simulink model "bpsk_cdm_carrier_lpf_waveform"  (R2025b)
settings: Solver=FixedStepAuto  StartTime=0.0  StopTime=50/6.2e6  MaxStep=3.33e-9  RelTol=1e-3
undefined symbols (not defined in the file): K, wc
libraries: commseqgen3 x4, commfilt2 x3, dspstat3 x2, commchan3 x1, commdigbbndpm3 x1, commrandsrc3 x1
settings Model: Creator=trish  LastModifiedBy=axolotl

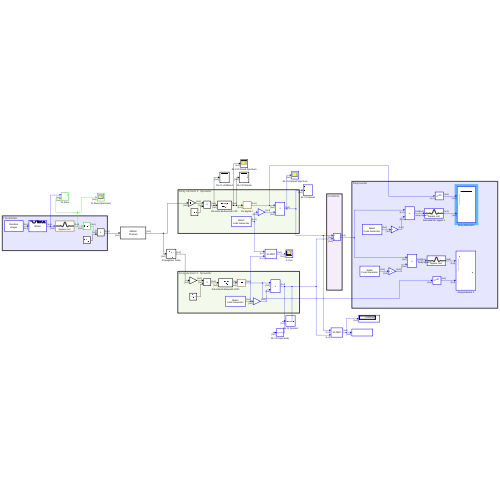
[thumbnail: Simulink's stored preview of the top-level diagram]
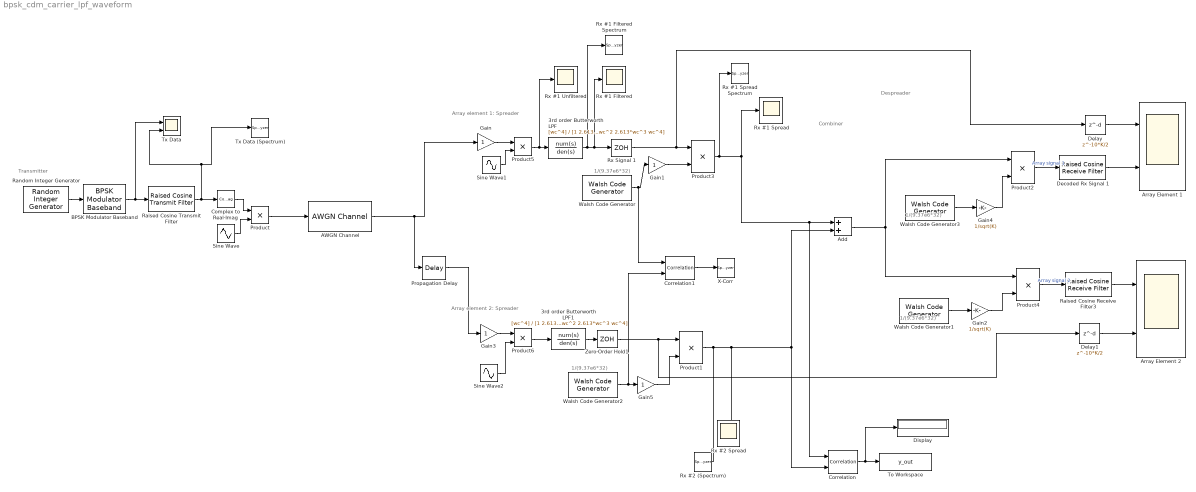
== system bpsk_cdm_carrier_lpf_waveform ==
  note: Despreader
  note: Combiner
  note: 1/(9.37e6*32)
  note: Array element 1: Spreader
  note: Transmitter
  note: 1/(9.37e6*32)
  note: 1/(9.37e6*32)
  note: Array element 2: Spreader
  note: 1/(9.37e6*32)
  3rd order Butterworth LPF : TransferFcn  Numerator=[wc^4]  Denominator=[1 2.613*wc 3.414*wc^2 2.613*wc^3 wc^4]
  3rd order Butterworth LPF1 : TransferFcn  Numerator=[wc^4]  Denominator=[1 2.613*wc 3.414*wc^2 2.613*wc^3 wc^4]
  AWGN Channel : commchan3/AWGN Channel  LegacyMode=off  NoiseMethod="Signal to noise ratio  (SNR)"  noiseMode="Signal to noise ratio  (SNR)"  EbNo=10  EsNo=10  SNR=10  BitsPerSymbol=1  SignalPower=1  SpecifySymbolPeriod=off  SamplesPerSymbol=1  SymbolPeriod=1  VarianceSource=Parameter  Variance=1  RandomStream=mt19937ar with seed  Seed=67  SimulateUsing=Code generation
  Add : Sum
  Array Element 1 : Scope  NumInputPorts=2
      settings: ActiveDisplayYMinimum=-0.22565656393453695  ActiveDisplayYMaximum=0.20472975996592438  DataLoggingVariableName=ScopeData7
  Array Element 2 : Scope  NumInputPorts=2
      settings: TimeUnits=Metric (based on Time Span)  ActiveDisplayYMinimum=-0.25790948055422058  ActiveDisplayYMaximum=0.25862522470755545  YLabel=Amplitude  DataLoggingVariableName=ScopeData2
  BPSK Modulator Baseband : commdigbbndpm3/BPSK Modulator Baseband  Ph=0  outDtype=double  outWordLen=16  outUDDataType=sfix(16)  outFracLenMode=Best precision  outFracLen=15  outDataTypeStr=double  outLastDataTypeStr=double
  Complex to Real-Imag : ComplexToRealImag  Output=Real
  Correlation : dspstat3/Correlation  domain=Time  roundingMode=Floor  overflowMode=off  outputDataTypeStr=Inherit: Same as accumulator  outputMin=[]  outputMax=[]  outputLastDataTypeStr=Inherit: Same as accumulator
  Correlation1 : dspstat3/Correlation  domain=Time  roundingMode=Floor  overflowMode=off  outputDataTypeStr=Inherit: Same as accumulator  outputMin=[]  outputMax=[]  outputLastDataTypeStr=Inherit: Same as accumulator
  Decoded Rx Signal 1 : commfilt2/Raised Cosine Receive Filter  filtType=Square root  R=0.5  filtSpan=10  N=K  downFactor=1  downOffset=0  filterGain=1  RateOptions=Allow multirate processing  framing=Mute  checkCoeff=off  variableName=rcRxFilt2  currentFiltSpan=10  D=5  inputOffset=0  sampMode=Mute  saveAsFlag=0  rateMode=Downsampling  checkGain=Normalized  launchFVT=on  roundingMode=Floor  overflowMode=off  coeffDataTypeStr=Inherit: Same word length as input  coeffMin=[]  coeffMax=[]  coeffLastDataTypeStr=Inherit: Same word length as input  accumDataTypeStr=Inherit: Same as product output  accumLastDataTypeStr=Inherit: Same as product output  outputDataTypeStr=Inherit: Same as accumulator  outputMin=[]  outputMax=[]  outputLastDataTypeStr=Inherit: Same as accumulator
  Delay : Delay  DelayLength=10*K/2
  Delay1 : Delay  DelayLength=10*K/2
  Display : Display
  Gain{,1,3,5} (4 alike) : Gain
  Gain2 : Gain  Gain=1/sqrt(K)
  Gain4 : Gain  Gain=1/sqrt(K)
  Product{,1..6} (7 alike) : Product
  Propagation Delay : TransportDelay  DelayTime=2e-9  TransDelayFeedthrough=on
  Raised Cosine Receive Filter3 : commfilt2/Raised Cosine Receive Filter  filtType=Square root  R=0.5  filtSpan=10  N=K  downFactor=1  downOffset=0  filterGain=1  RateOptions=Allow multirate processing  framing=Mute  checkCoeff=off  variableName=rcRxFilt3  currentFiltSpan=10  D=5  inputOffset=0  sampMode=Mute  saveAsFlag=0  rateMode=Downsampling  checkGain=Normalized  launchFVT=on  roundingMode=Floor  overflowMode=off  coeffDataTypeStr=Inherit: Same word length as input  coeffMin=[]  coeffMax=[]  coeffLastDataTypeStr=Inherit: Same word length as input  accumDataTypeStr=Inherit: Same as product output  accumLastDataTypeStr=Inherit: Same as product output  outputDataTypeStr=Inherit: Same as accumulator  outputMin=[]  outputMax=[]  outputLastDataTypeStr=Inherit: Same as accumulator
  Raised Cosine Transmit Filter : commfilt2/Raised Cosine Transmit Filter  filtType=Square root  R=0.5  filtSpan=10  N=K*5  filterGain=1  RateOptions=Allow multirate processing  framing=Mute  checkCoeff=off  variableName=rcTxFilt  checkGain=Normalized  sampMode=Mute  saveAsFlag=0  currentFiltSpan=10  D=5  launchFVT=on  roundingMode=Floor  overflowMode=off  coeffDataTypeStr=Inherit: Same word length as input  coeffMin=[]  coeffMax=[]  coeffLastDataTypeStr=Inherit: Same word length as input  outputDataTypeStr=Inherit: Same as accumulator  outputMin=[]  outputMax=[]  outputLastDataTypeStr=Inherit: Same as accumulator
      settings: LibrarySourceBlock=|
      | commhdlfilt/Raised Cosine
      | Transmit Filter
  Random Integer Generator : commrandsrc3/Random Integer Generator  SetSize=2  SeedSource=Parameter  Seed=32  SampleTime=1/(6.25e6)  SamplesPerFrame=1  OutputDataType=single  SimulateUsing=Interpreted execution
  Rx #1 Filtered : Scope
      settings: TimeUnits=Metric (based on Time Span)  ActiveDisplayYMinimum=-0.50683787517471779  ActiveDisplayYMaximum=0.55095946181705846  YLabel=Amplitude  DataLoggingVariableName=ScopeData4
  Rx #1 Filtered Spectrum : SpectrumAnalyzer  WindowPosition=[133.000000,75.000000,2748.000000,1782.000000,]  ScopeFrameLocation=window  SpectrumType=Power density  Method=Welch  WindowInvariantSamplesPerUpdate=on  Span=300e6  StartFrequency=-25000000  StopFrequency=25000000  SpectrumUnits=dBm/Hz  YLimits=[-331.5621 29.6853]  ExpandToolstrip=on  SelectedToolstripTab=spectrumAnalyzerToolstrip.estimationTab
      settings: OpenAtSimulationStart=off
  Rx #1 Spread : Scope
      settings: TimeUnits=Metric (based on Time Span)  ActiveDisplayYMinimum=-0.38058083882507643  ActiveDisplayYMaximum=0.3711759796363393  YLabel=Amplitude  DataLoggingVariableName=ScopeData3
  Rx #1 Spread Spectrum : SpectrumAnalyzer  WindowPosition=[89.000000,50.000000,1832.000000,1188.000000,]  ScopeFrameLocation=window  SpectrumType=Power density  Method=Welch  WindowInvariantSamplesPerUpdate=on  Span=300e6  StartFrequency=-25000000  StopFrequency=25000000  SpectrumUnits=dBm/Hz  YLimits=[-148.08026488239346 -43.11631661926841]  ExpandToolstrip=on  SelectedToolstripTab=spectrumAnalyzerToolstrip.estimationTab
      settings: OpenAtSimulationStart=off
  Rx #1 Unfiltered : Scope
      settings: TimeUnits=Metric (based on Time Span)  ActiveDisplayYMinimum=-4.3884399589650158  ActiveDisplayYMaximum=5.1372737935889194  YLabel=Amplitude  DataLoggingVariableName=ScopeData6
  Rx #2 (Spectrum) : SpectrumAnalyzer  WindowPosition=[149.000000,75.000000,2732.000000,1782.000000,]  ScopeFrameLocation=window  SpectrumType=Power density  Method=Welch  WindowInvariantSamplesPerUpdate=on  Span=300e6  StartFrequency=-25000000  StopFrequency=25000000  SpectrumUnits=dBm/Hz  YLimits=[-151.3459 -44.247]  ExpandToolstrip=on  SelectedToolstripTab=spectrumAnalyzerToolstrip.estimationTab
      settings: OpenAtSimulationStart=off
  Rx #2 Spread : Scope
      settings: TimeUnits=Metric (based on Time Span)  ActiveDisplayYMinimum=-0.38058083882507643  ActiveDisplayYMaximum=0.3711759796363393  YLabel=Amplitude
  Rx Signal 1 : ZeroOrderHold  SampleTime=1/(K*9.35e6)
  Sine Wave : Sin  Frequency=2*pi*500e6  Phase=pi/2  SampleTime=0
  Sine Wave1 : Sin  Frequency=2*pi*500e6  Phase=pi/2  SampleTime=0
  Sine Wave2 : Sin  Frequency=2*pi*500e6  Phase=pi/2  SampleTime=0
  To Workspace : ToWorkspace  VariableName=y_out  SampleTime=-1
      settings: Save2DSignal=2-D array (concatenate along first dimension)
  Tx Data : Scope  NumInputPorts=2
      settings: ActiveDisplayYMinimum=-1.25  ActiveDisplayYMaximum=1.25
  Tx Data (Spectrum) : SpectrumAnalyzer  WindowPosition=[4261.000000,672.000000,1832.000000,1188.000000,]  ScopeFrameLocation=window  SpectrumType=Power density  Method=Welch  WindowInvariantSamplesPerUpdate=on  Span=60e6  StartFrequency=-25000000  StopFrequency=25000000  SpectrumUnits=dBm/Hz  YLimits=[-129.66030778637997 -44.78293119034885]  ExpandToolstrip=on  SelectedToolstripTab=spectrumAnalyzerToolstrip.estimationTab
      settings: OpenAtSimulationStart=off
  Walsh Code Generator : commseqgen3/Walsh Code Generator  Length=K  Index=1  SampleTime=1/(K*9.35e6)  SamplesPerFrame=1  OutputDataType=int8  SimulateUsing=Code generation
  Walsh Code Generator1 : commseqgen3/Walsh Code Generator  Length=K  Index=2  SampleTime=1/(K*9.35e6)  SamplesPerFrame=1  OutputDataType=double  SimulateUsing=Code generation
  Walsh Code Generator2 : commseqgen3/Walsh Code Generator  Length=K  Index=2  SampleTime=1/(K*9.35e6)  SamplesPerFrame=1  OutputDataType=int8  SimulateUsing=Code generation
  Walsh Code Generator3 : commseqgen3/Walsh Code Generator  Length=K  Index=1  SampleTime=1/(K*9.35e6)  SamplesPerFrame=1  OutputDataType=double  SimulateUsing=Code generation
  X-Corr : SpectrumAnalyzer  WindowPosition=[3520.000000,578.000000,1832.000000,1188.000000,]  ScopeFrameLocation=window  SpectrumType=Power density  Method=Welch  WindowInvariantSamplesPerUpdate=on  Span=300e6  StartFrequency=-25000000  StopFrequency=25000000  SpectrumUnits=dBW/Hz  ReferenceLoad=50  YLimits=[-4880.211409223666 2317.2443220767536]  ExpandToolstrip=on  SelectedToolstripTab=spectrumAnalyzerToolstrip.measurementsTab
      settings: OpenAtSimulationStart=off
  Zero-Order Hold1 : ZeroOrderHold  SampleTime=1/(K*9.35e6)
  wires:
  Gain1/1 -> Product3/2
  Walsh Code Generator/1 -> Correlation1/1, Gain1/1
  Random Integer Generator/1 -> BPSK Modulator Baseband/1
  Walsh Code Generator1/1 -> Gain2/1
  Walsh Code Generator3/1 -> Gain4/1
  Gain4/1 -> Product2/2
  Add/1 -> Product4/1, Product2/1
  Product2/1 -> Decoded Rx Signal 1/1  "Array signal 1"
  Product4/1 -> Raised Cosine Receive Filter3/1  "Array signal 2"
  Raised Cosine Receive Filter3/1 -> Array Element 2/1
  Gain2/1 -> Product4/2
  Raised Cosine Transmit Filter/1 -> Complex to Real-Imag/1, Tx Data (Spectrum)/1, Tx Data/2
  BPSK Modulator Baseband/1 -> Tx Data/1, Raised Cosine Transmit Filter/1
  Rx Signal 1/1 -> Delay/1, Product3/1
  Propagation Delay/1 -> Gain3/1
  Zero-Order Hold1/1 -> Delay1/1, Product1/1
  Walsh Code Generator2/1 -> Correlation1/2, Gain5/1
  Gain5/1 -> Product1/2
  Correlation/1 -> Display/1, To Workspace/1
  Product3/1 -> Rx #1 Spread Spectrum/1, Correlation/1, Add/1, Rx #1 Spread/1
  Product1/1 -> Rx #2 (Spectrum)/1, Add/2, Correlation/2, Rx #2 Spread/1
  Sine Wave/1 -> Product/2
  Complex to Real-Imag/1 -> Product/1
  Product/1 -> AWGN Channel/1
  Sine Wave1/1 -> Product5/2
  Gain/1 -> Product5/1
  3rd order Butterworth LPF/1 -> Rx #1 Filtered/1, Rx Signal 1/1, Rx #1 Filtered Spectrum/1
  AWGN Channel/1 -> Propagation Delay/1, Gain/1
  Product5/1 -> Rx #1 Unfiltered/1, 3rd order Butterworth LPF/1
  Decoded Rx Signal 1/1 -> Array Element 1/2
  Delay/1 -> Array Element 1/1
  Sine Wave2/1 -> Product6/2
  Gain3/1 -> Product6/1
  3rd order Butterworth LPF1/1 -> Zero-Order Hold1/1
  Product6/1 -> 3rd order Butterworth LPF1/1
  Delay1/1 -> Array Element 2/2
  Correlation1/1 -> X-Corr/1
